simulink model "test_codegen_sim_02"  (Simulink 7.9)
settings: Solver=ode45  StartTime=0.0  StopTime=10.0  RelTol=1e-3
libraries: mpt_sim x1
settings Model: Creator=mato  LastModifiedBy=mato

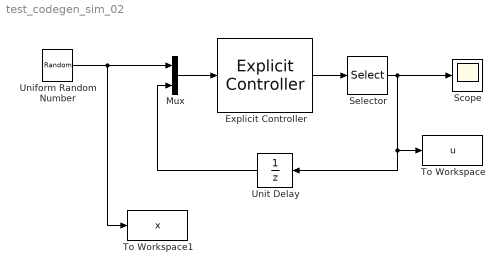
== system test_codegen_sim_02 ==
  Explicit Controller : mpt_sim/Explicit Controller
  Mux : Mux  Inputs=2
  Scope : Scope
      settings: TimeRange=10
  Selector : Selector  InputPortWidth=3  IndexOptions=Index vector (dialog)  Indices=1  OutputSizes=1
  To Workspace : ToWorkspace  VariableName=u  SampleTime=-1
  To Workspace1 : ToWorkspace  VariableName=x  SampleTime=-1
  Uniform Random Number : UniformRandomNumber  Seed=[0;1]  SampleTime=1
  Unit Delay : UnitDelay  SampleTime=-1
  wires:
  Explicit Controller/1 -> Selector/1
  Uniform Random Number/1 -> To Workspace1/1, Mux/1
  Mux/1 -> Explicit Controller/1
  Unit Delay/1 -> Mux/2
  Selector/1 -> Scope/1, To Workspace/1, Unit Delay/1
